simulink model "Rotary_inverted_pendulum_simscape_model"  (R2026b)
settings: Solver=VariableStepAuto  StopTime=10  EnableMultiTasking=on
InitFcn:
  | Rotary_inverted_pendulum_params;
values from neighbouring files (symbols this model uses):
  A = [0 0 1.58599833727e-11 -4.90689813272e-13 0 0 11.773740367 153.017565535 1 0 -0.668730280726 -0.988272810616 ... (16 elements, 4x4)]    [Rotary_inverted_pendulum_control_.mat]    (also in Rotary_inverted_pendulum_params.m = A_hand; Rotary_inverted_pendulum_symbolic.m = zeros(4,4))
  alpha_0 = 170    [Rotary_inverted_pendulum_params.m]
  alpha_cal = -3.678    [Rotary_inverted_pendulum_params.m]
  B = [0 0 3.48321726757 5.14775001613]    [Rotary_inverted_pendulum_control_.mat]    (also in Rotary_inverted_pendulum_params.m = B_hand; Rotary_inverted_pendulum_symbolic.m = zeros(4,1))
  C = [1 0 0 0; 0 1 0 0]    [Rotary_inverted_pendulum_params.m]
  D = [0; 0]    [Rotary_inverted_pendulum_params.m]
  K_c = place(A,B,[-8 -5 -6 -1])    [Rotary_inverted_pendulum_params.m]
  km = 0.035    [Rotary_inverted_pendulum_params.m]
  kt = 0.035    [Rotary_inverted_pendulum_params.m]
  L = 264e-6    (= 0.000264)    [Rotary_inverted_pendulum_params.m]
  L_o = place(A',C',5*[-8 -5 -6 -1])'    [Rotary_inverted_pendulum_params.m]
  link_mass = 0.08    [Rotary_inverted_pendulum_params.m]
  N = 1    [Rotary_inverted_pendulum_params.m]
  p_mass = 0.1    [Rotary_inverted_pendulum_params.m]
  R = 7.14    [Rotary_inverted_pendulum_params.m]    (also in Rotary_inverted_pendulum_symbolic.m = 2)
  rod_mass = 0.05    [Rotary_inverted_pendulum_params.m]
  rt1 = 7/2    (= 3.5)    [Rotary_inverted_pendulum_params.m]
  rt2 = 8.5-0.4    (= 8.1)    [Rotary_inverted_pendulum_params.m]
  V_max = 24    [Rotary_inverted_pendulum_params.m]
undefined symbols (not defined in the file or in its folder): K, L_q, X, Y, Z
libraries: sm_lib x123, nesl_utility x29, simulink x10
(part 1 of 4)
settings Model: Creator=ControlLab2  LastModifiedBy=Mrsh
settings DataIOCC: LimitDataPoints=on  MaxDataPoints=10000
settings OptimizationCC: LifeSpan=inf
settings DebuggingCC: AllowSymbolicDim=off  ArithmeticOperatorsInVariantConditions=warning  SFExecutionAtInitializationDiag=none  SFNoUnconditionalDefaultTransitionDiag=warning  SFUnexpectedBacktrackingDiag=warning
settings SFSimCC: CustomCodeUndefinedFunction=UseInterfaceOnly  SimUseLocalCustomCode=off
settings RTWCC: RTWUseLocalCustomCode=off
settings CodeAppCC: StateflowObjectComments=on
settings GRTTargetCC: TargetLangStandard=C89/C90 (ANSI)
settings ConfigComp: CovExternalEMLEnable=off  CovSFcnEnable=off  CovSaveCumulativeToWorkspaceVar=on  CovSaveSingleToWorkspaceVar=on
settings SimscapeCC: SimscapeLogSimulationStatistics=on  SimscapeLogType=all  SimscapeUseEnergyAccounting=off
settings ExplorerConfigSet: InternalSimMechanicsExplorerSettings=|
  | <ExplorerConfiguration>
  | 
  |   <canonicalview>default</canonicalview>
  | 
  |   <TilePanel>
  |     <TileInfo>
  |       <Tiles Columns="1" Count="1" Height="610" Rows="1" Width="1088">
  |         <Row Weight="1"/>
  |         <Column Weight="1"/>
  |         <Tile Height="1" Width="1" X="0" Y="0"/>
  |       </Tiles>
  |     </TileInfo>
  |     <SceneInfo>
  |       <SceneViewer>
  |         <IsThisViewStd>
  |           <IsStandardView>off</IsStandardView>
  |           <StandardViewName>Front</StandardViewName>
  |         </IsThisViewStd>
  |         <BGColor>
  |           <R>1</R>
  |           <G>1</G>
  |           <B>1</B>
  |           <A>1</A>
  |         </BGColor>
  |         <Camera>
  |           <DoPerspective>off</DoPerspective>
  |           <Position>
  |             <X>0.705670544528059</X>
  |             <Y>-0.69361970210692636</Y>
  |             <Z>0.40320052935287365</Z>
  |           </Position>
  |           <Center>
  |             <X>0.05090138860052084</X>
  |             <Y>-0.026375091476912745</Y>
  |             <Z>0.0012447022565247549</Z>
  |           </Center>
  |           <Up>
  |             <X>-0.2787747011801574</X>
  |             <Y>0.27985805213160481</Y>
  |             <Z>0.91867520737147246</Z>
  |           </Up>
  |           <XLim>0.14182089495266087</XLim>
  |           <YLim>0.14182089495266087</YLim>
  |           <ViewLimDist>0.01</ViewLimDist>
  |         </Camera>
  |       </SceneViewer>
  |     </SceneInfo>
  |   </TilePanel>
  | 
  |   <MechEditorPanel>
  |     <GfxPanelCameraMap/>
  |     <Cameras/>
  |     <VideoCreator>
  |       <IncludeTiles>All</IncludeTiles>
  |       <IncludeTime>on</IncludeTime>
  |       <IncludeWorldFrame>off</IncludeWorldFrame>
  |       <PlaybackSpeedRatio>1</PlaybackSpeedRatio>
  |       <FrameRate>30</FrameRate>
  |       <FrameSize>auto</FrameSize>
  |       <VideoFormat>MotionJPEGAVI</VideoFormat>
  |     </VideoCreator>
  |   </MechEditorPanel>
  | 
  |   <PlaybackSettings>
  |     <PlaybackSpeedFactor>1</PlaybackSpeedFactor>
  |   </PlaybackSettings>
  | 
  | </ExplorerConfiguration>

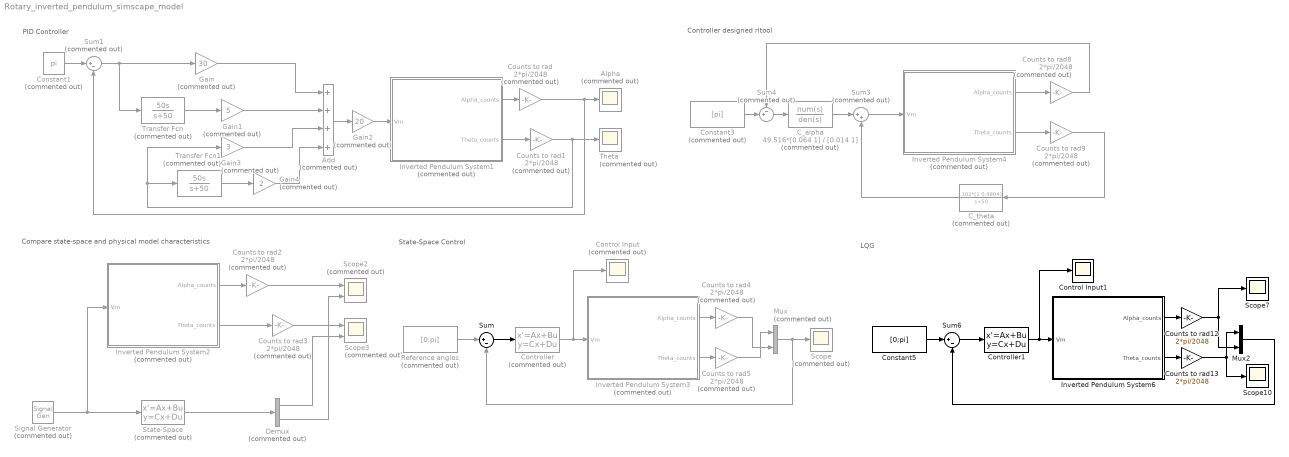
== system Rotary_inverted_pendulum_simscape_model ==
  note: PID Controller
  note: Compare state-space and physical model characteristics
  note: Controller designed rltool
  note: State-Space Control
  note: LQG
  Add : Sum  Commented=on  Inputs=++++
  Alpha : Scope  Commented=on
      settings: ActiveDisplayYMinimum=3.02651  ActiveDisplayYMaximum=3.22203
  C_alpha : TransferFcn  Commented=on  Numerator=49.516*[0.064 1]  Denominator=[0.014 1]
  C_theta : TransferFcn  Commented=on  Numerator=102*[1 0.9804]  Denominator=[1 50]
  Constant1 : Constant  Commented=on  Value=pi
  Constant3 : Constant  Commented=on  Value=[pi]
  Constant5 : Constant  Value=[0;pi]
  Control Input : Scope  Commented=on
      settings: ActiveDisplayYMinimum=-33.02101  ActiveDisplayYMaximum=31.32481
  Control Input1 : Scope
      settings: ActiveDisplayYMinimum=-7.48608  ActiveDisplayYMaximum=18.51296  DataLoggingVariableName=ULog  DataLoggingSaveFormat=Array
  Controller : StateSpace  Commented=on  A=A-B*K_c-L_o*C  B=L_o  C=K_c  D=[0 0]  InitialCondition=0
  Controller1 : StateSpace  A=A-B*K-L_q*C  B=L_q  C=K  D=[0 0]  InitialCondition=0
  Counts to rad{,1..5,8..9} (8 alike) : Gain  Commented=on  Gain=2*pi/2048
  Counts to rad12 : Gain  Gain=2*pi/2048
  Counts to rad13 : Gain  Gain=2*pi/2048
  Demux : Demux  Commented=on  Outputs=2
  Gain : Gain  Commented=on  Gain=30
  Gain1 : Gain  Commented=on  Gain=5
  Gain2 : Gain  Commented=on  Gain=20
  Gain3 : Gain  Commented=on  Gain=3
  Gain4 : Gain  Commented=on  Gain=2
  Inverted Pendulum System1 : Subsystem  Commented=on  mask{kt=kt, km=km, R=R, L=L, alpha_0=175}
      mask prompts: kt "Torque constant (Nm/A)"; km "Back EMF constant (V/(rad/s))"; R "Resistance (Ohm)"; L "Inductance (H)"; alpha_0 "Pendulum initial angle (deg)"
      mask init:
      | % Inverted Pendulum Parameters
      | base_size=7;%cm
      | rod_rad=1;
      | rod_length=8.5;
      | rod_mass=0.095;
      | p_rad=1;
      | p_length=12.9;
      | p_mass=0.024;
      | rt1=base_size/2;
      | rt2=rod_length-0.4;
      | rt4=p_length/2;
      | D_r=0.0015/2;
      | D_p=0.0005/2;
  Inverted Pendulum System2 : Subsystem  Commented=on  mask{kt=kt, km=km, R=R, L=L, alpha_0=0}
      mask prompts: kt "Torque constant (Nm/A)"; km "Back EMF constant (V/(rad/s))"; R "Resistance (Ohm)"; L "Inductance (H)"; alpha_0 "Pendulum initial angle (deg)"
      mask init: same as Rotary_inverted_pendulum_simscape_model/Inverted Pendulum System1
  Inverted Pendulum System3 : Subsystem  Commented=on  mask{kt=kt, km=km, R=R, L=L, alpha_0=165}
      mask prompts: kt "Torque constant (Nm/A)"; km "Back EMF constant (V/(rad/s))"; R "Resistance (Ohm)"; L "Inductance (H)"; alpha_0 "Pendulum initial angle (deg)"
      mask init: same as Rotary_inverted_pendulum_simscape_model/Inverted Pendulum System1
  Inverted Pendulum System4 : Subsystem  Commented=on  mask{kt=kt, km=km, R=R, L=L, alpha_0=175}
      mask prompts: kt "Torque constant (Nm/A)"; km "Back EMF constant (V/(rad/s))"; R "Resistance (Ohm)"; L "Inductance (H)"; alpha_0 "Pendulum initial angle (deg)"
      mask init: same as Rotary_inverted_pendulum_simscape_model/Inverted Pendulum System1
  Inverted Pendulum System6 : Subsystem  mask{kt=kt, km=km, R=R, L=L, alpha_0=alpha_0}
      mask prompts: kt "Torque constant (Nm/A)"; km "Back EMF constant (V/(rad/s))"; R "Resistance (Ohm)"; L "Inductance (H)"; alpha_0 "Pendulum initial angle (deg)"
      mask init:
      | % All parameters come from Rotary_inverted_pendulum_realistic_params.m
  Mux : Mux  Commented=on  Inputs=2
  Mux2 : Mux  Inputs=2
  Reference angles : Constant  Commented=on  Value=[0;pi]
  Scope : Scope  Commented=on
      settings: ActiveDisplayYMinimum=-0.50694  ActiveDisplayYMaximum=3.69747  DataLoggingVariableName=ScopeData3
  Scope10 : Scope
      settings: ActiveDisplayYMinimum=-0.24263  ActiveDisplayYMaximum=1.50161  DataLoggingVariableName=ThetaLog  DataLoggingSaveFormat=Array
  Scope2 : Scope  Commented=on  NumInputPorts=2
      settings: ActiveDisplayYMinimum=-4.48254  ActiveDisplayYMaximum=4.62282  DataLoggingVariableName=ScopeData2
  Scope3 : Scope  Commented=on  NumInputPorts=2
      settings: ActiveDisplayYMinimum=-8.30374  ActiveDisplayYMaximum=0.94912  DataLoggingVariableName=ScopeData3
  Scope7 : Scope
      settings: ActiveDisplayYMinimum=2.818  ActiveDisplayYMaximum=3.3143  DataLoggingVariableName=AlphaLog  DataLoggingSaveFormat=Array
  Signal Generator : SignalGenerator  Commented=on  WaveForm=square
  State-Space : StateSpace  Commented=on  A=A  B=B  C=C  D=D  InitialCondition=0
  Sum : Sum  Inputs=|+-
  Sum1 : Sum  Commented=on  Inputs=|+-
  Sum3 : Sum  Commented=on  Inputs=|++
  Sum4 : Sum  Commented=on  Inputs=-+|
  Sum6 : Sum  Inputs=|+-
  Theta : Scope  Commented=on
      settings: ActiveDisplayYMinimum=-0.10248  ActiveDisplayYMaximum=0.25695  DataLoggingVariableName=ScopeData2
  Transfer Fcn : TransferFcn  Commented=on  Numerator=[50 0]  Denominator=[1 50]
  Transfer Fcn1 : TransferFcn  Commented=on  Numerator=[50 0]  Denominator=[1 50]
  wires:
  Constant1/1 -> Sum1/1
  Inverted Pendulum System1/1(Alpha_counts) -> Counts to rad/1
  Transfer Fcn/1 -> Gain1/1
  Transfer Fcn1/1 -> Gain4/1
  Inverted Pendulum System1/2(Theta_counts) -> Counts to rad1/1
  Gain/1 -> Add/1
  Gain1/1 -> Add/2
  Gain3/1 -> Add/3
  Gain4/1 -> Add/4
  Add/1 -> Gain2/1
  Signal Generator/1 -> Inverted Pendulum System2/1(Vm), State-Space/1
  Sum1/1 -> Transfer Fcn/1, Gain/1
  Inverted Pendulum System2/1(Alpha_counts) -> Counts to rad2/1
  Inverted Pendulum System2/2(Theta_counts) -> Counts to rad3/1
  Gain2/1 -> Inverted Pendulum System1/1(Vm)
  State-Space/1 -> Demux/1
  Demux/1 -> Scope3/2
  Demux/2 -> Scope2/2
  Reference angles/1 -> Sum/1
  Sum/1 -> Controller/1
  Mux/1 -> Scope/1, Sum/2
  Inverted Pendulum System3/2(Theta_counts) -> Counts to rad5/1
  Inverted Pendulum System3/1(Alpha_counts) -> Counts to rad4/1
  Counts to rad/1 -> Alpha/1, Sum1/2
  Counts to rad1/1 -> Theta/1, Transfer Fcn1/1, Gain3/1
  Counts to rad2/1 -> Scope2/1
  Counts to rad3/1 -> Scope3/1
  Counts to rad4/1 -> Mux/2
  Counts to rad5/1 -> Mux/1
  Controller/1 -> Inverted Pendulum System3/1(Vm), Control Input/1
  Inverted Pendulum System4/2(Theta_counts) -> Counts to rad9/1
  Inverted Pendulum System4/1(Alpha_counts) -> Counts to rad8/1
  C_theta/1 -> Sum3/2
  Counts to rad9/1 -> C_theta/1
  Constant3/1 -> Sum4/2
  Counts to rad8/1 -> Sum4/1
  Sum4/1 -> C_alpha/1
  C_alpha/1 -> Sum3/1
  Sum3/1 -> Inverted Pendulum System4/1(Vm)
  Controller1/1 -> Inverted Pendulum System6/1(Vm), Control Input1/1
  Constant5/1 -> Sum6/1
  Mux2/1 -> Sum6/2
  Inverted Pendulum System6/2(Theta_counts) -> Counts to rad13/1
  Inverted Pendulum System6/1(Alpha_counts) -> Counts to rad12/1
  Sum6/1 -> Controller1/1
  Counts to rad13/1 -> Scope10/1, Mux2/1
  Counts to rad12/1 -> Scope7/1, Mux2/2

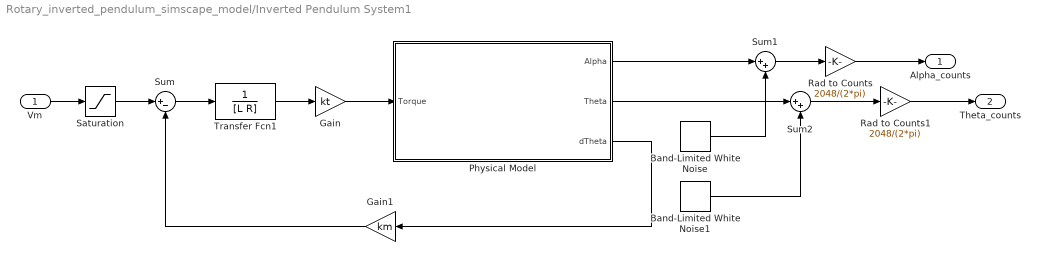
== system Rotary_inverted_pendulum_simscape_model/Inverted Pendulum System1 ==
  Vm : Inport
  Band-Limited White Noise : simulink/Sources/Band-Limited White Noise  Cov=[0.0000001]  Ts=0.001  seed=[23341]
  Band-Limited White Noise1 : simulink/Sources/Band-Limited White Noise  Cov=[0.0000001]  Ts=0.001  seed=[23341]
  Gain : Gain  Gain=kt
  Gain1 : Gain  Gain=km
  Physical Model : Subsystem
  Rad to Counts : Gain  Gain=2048/(2*pi)
  Rad to Counts1 : Gain  Gain=2048/(2*pi)
  Saturation : Saturate  UpperLimit=10  LowerLimit=-10
  Sum : Sum  Inputs=|+-
  Sum1 : Sum  Inputs=|++
  Sum2 : Sum  Inputs=|++
  Transfer Fcn1 : TransferFcn  Denominator=[L R]
  Alpha_counts : Outport
  Theta_counts : Outport  Port=2
  wires:
  Saturation/1 -> Sum/1
  Rad to Counts1/1 -> Theta_counts/1
  Rad to Counts/1 -> Alpha_counts/1
  Band-Limited White Noise1/1 -> Sum2/2
  Band-Limited White Noise/1 -> Sum1/2
  Sum2/1 -> Rad to Counts1/1
  Sum1/1 -> Rad to Counts/1
  Sum/1 -> Transfer Fcn1/1
  Transfer Fcn1/1 -> Gain/1
  Gain1/1 -> Sum/2
  Physical Model/3(dTheta) -> Gain1/1
  Gain/1 -> Physical Model/1(Torque)
  Vm/1 -> Saturation/1
  Physical Model/1(Alpha) -> Sum1/1
  Physical Model/2(Theta) -> Sum2/1

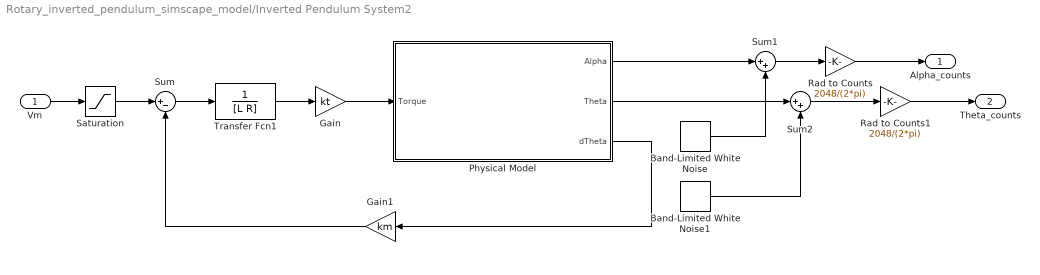
== system Rotary_inverted_pendulum_simscape_model/Inverted Pendulum System2 ==
  Vm : Inport
  Band-Limited White Noise : simulink/Sources/Band-Limited White Noise  Cov=[0.0000001]  Ts=0.001  seed=[23341]
  Band-Limited White Noise1 : simulink/Sources/Band-Limited White Noise  Cov=[0.0000001]  Ts=0.001  seed=[23341]
  Gain : Gain  Gain=kt
  Gain1 : Gain  Gain=km
  Physical Model : Subsystem
  Rad to Counts : Gain  Gain=2048/(2*pi)
  Rad to Counts1 : Gain  Gain=2048/(2*pi)
  Saturation : Saturate  UpperLimit=10  LowerLimit=-10
  Sum : Sum  Inputs=|+-
  Sum1 : Sum  Inputs=|++
  Sum2 : Sum  Inputs=|++
  Transfer Fcn1 : TransferFcn  Denominator=[L R]
  Alpha_counts : Outport
  Theta_counts : Outport  Port=2
  wires:
  Saturation/1 -> Sum/1
  Rad to Counts1/1 -> Theta_counts/1
  Rad to Counts/1 -> Alpha_counts/1
  Band-Limited White Noise1/1 -> Sum2/2
  Band-Limited White Noise/1 -> Sum1/2
  Sum2/1 -> Rad to Counts1/1
  Sum1/1 -> Rad to Counts/1
  Sum/1 -> Transfer Fcn1/1
  Transfer Fcn1/1 -> Gain/1
  Gain1/1 -> Sum/2
  Physical Model/3(dTheta) -> Gain1/1
  Gain/1 -> Physical Model/1(Torque)
  Vm/1 -> Saturation/1
  Physical Model/1(Alpha) -> Sum1/1
  Physical Model/2(Theta) -> Sum2/1

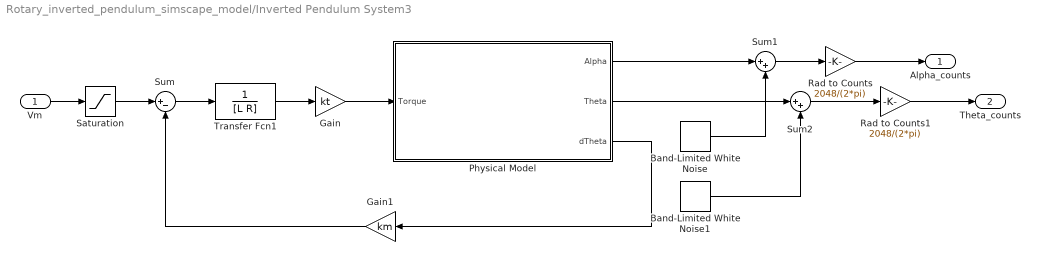
== system Rotary_inverted_pendulum_simscape_model/Inverted Pendulum System3 ==
  Vm : Inport
  Band-Limited White Noise : simulink/Sources/Band-Limited White Noise  Cov=[0.0000001]  Ts=0.001  seed=[23341]
  Band-Limited White Noise1 : simulink/Sources/Band-Limited White Noise  Cov=[0.0000001]  Ts=0.001  seed=[23341]
  Gain : Gain  Gain=kt
  Gain1 : Gain  Gain=km
  Physical Model : Subsystem
  Rad to Counts : Gain  Gain=2048/(2*pi)
  Rad to Counts1 : Gain  Gain=2048/(2*pi)
  Saturation : Saturate  UpperLimit=10  LowerLimit=-10
  Sum : Sum  Inputs=|+-
  Sum1 : Sum  Inputs=|++
  Sum2 : Sum  Inputs=|++
  Transfer Fcn1 : TransferFcn  Denominator=[L R]
  Alpha_counts : Outport
  Theta_counts : Outport  Port=2
  wires:
  Saturation/1 -> Sum/1
  Rad to Counts1/1 -> Theta_counts/1
  Rad to Counts/1 -> Alpha_counts/1
  Band-Limited White Noise1/1 -> Sum2/2
  Band-Limited White Noise/1 -> Sum1/2
  Sum2/1 -> Rad to Counts1/1
  Sum1/1 -> Rad to Counts/1
  Sum/1 -> Transfer Fcn1/1
  Transfer Fcn1/1 -> Gain/1
  Gain1/1 -> Sum/2
  Physical Model/3(dTheta) -> Gain1/1
  Gain/1 -> Physical Model/1(Torque)
  Vm/1 -> Saturation/1
  Physical Model/1(Alpha) -> Sum1/1
  Physical Model/2(Theta) -> Sum2/1

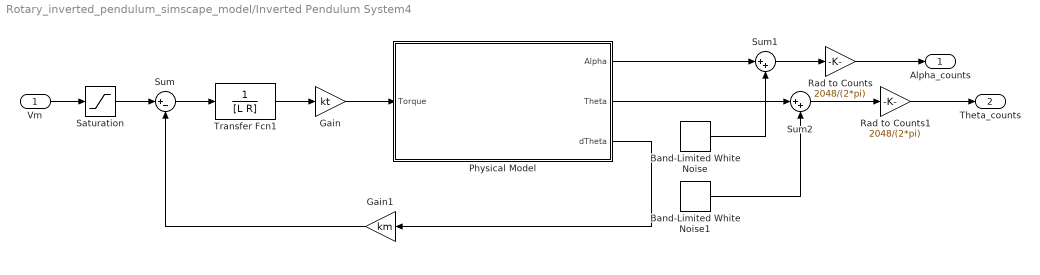
== system Rotary_inverted_pendulum_simscape_model/Inverted Pendulum System4 ==
  Vm : Inport
  Band-Limited White Noise : simulink/Sources/Band-Limited White Noise  Cov=[0.0000001]  Ts=0.001  seed=[23341]
  Band-Limited White Noise1 : simulink/Sources/Band-Limited White Noise  Cov=[0.0000001]  Ts=0.001  seed=[23341]
  Gain : Gain  Gain=kt
  Gain1 : Gain  Gain=km
  Physical Model : Subsystem
  Rad to Counts : Gain  Gain=2048/(2*pi)
  Rad to Counts1 : Gain  Gain=2048/(2*pi)
  Saturation : Saturate  UpperLimit=10  LowerLimit=-10
  Sum : Sum  Inputs=|+-
  Sum1 : Sum  Inputs=|++
  Sum2 : Sum  Inputs=|++
  Transfer Fcn1 : TransferFcn  Denominator=[L R]
  Alpha_counts : Outport
  Theta_counts : Outport  Port=2
  wires:
  Saturation/1 -> Sum/1
  Rad to Counts1/1 -> Theta_counts/1
  Rad to Counts/1 -> Alpha_counts/1
  Band-Limited White Noise1/1 -> Sum2/2
  Band-Limited White Noise/1 -> Sum1/2
  Sum2/1 -> Rad to Counts1/1
  Sum1/1 -> Rad to Counts/1
  Sum/1 -> Transfer Fcn1/1
  Transfer Fcn1/1 -> Gain/1
  Gain1/1 -> Sum/2
  Physical Model/3(dTheta) -> Gain1/1
  Gain/1 -> Physical Model/1(Torque)
  Vm/1 -> Saturation/1
  Physical Model/1(Alpha) -> Sum1/1
  Physical Model/2(Theta) -> Sum2/1

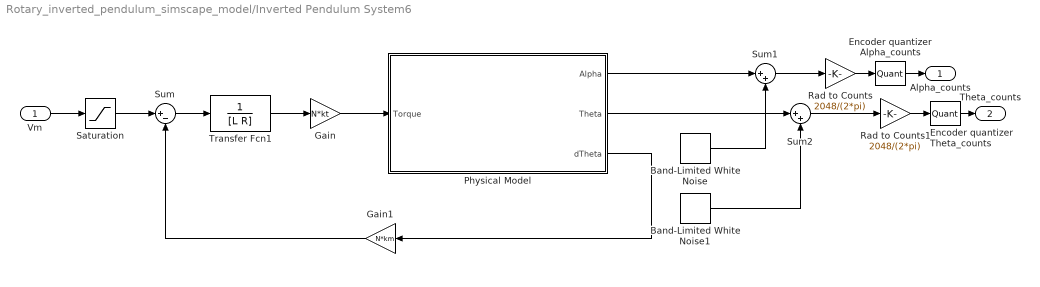
== system Rotary_inverted_pendulum_simscape_model/Inverted Pendulum System6 ==
  Vm : Inport
  Band-Limited White Noise : simulink/Sources/Band-Limited White Noise  Cov=[0.0000001]  Ts=0.001  seed=[23341]
  Band-Limited White Noise1 : simulink/Sources/Band-Limited White Noise  Cov=[0.0000001]  Ts=0.001  seed=[23341]
  Encoder quantizer Alpha_counts : Quantizer  QuantizationInterval=1
  Encoder quantizer Theta_counts : Quantizer  QuantizationInterval=1
  Gain : Gain  Gain=N*kt
  Gain1 : Gain  Gain=N*km
  Physical Model : Subsystem
  Rad to Counts : Gain  Gain=2048/(2*pi)
  Rad to Counts1 : Gain  Gain=2048/(2*pi)
  Saturation : Saturate  UpperLimit=V_max  LowerLimit=-V_max
  Sum : Sum  Inputs=|+-
  Sum1 : Sum  Inputs=|++
  Sum2 : Sum  Inputs=|++
  Transfer Fcn1 : TransferFcn  Denominator=[L R]
  Alpha_counts : Outport
  Theta_counts : Outport  Port=2
  wires:
  Saturation/1 -> Sum/1
  Band-Limited White Noise1/1 -> Sum2/2
  Band-Limited White Noise/1 -> Sum1/2
  Sum2/1 -> Rad to Counts1/1
  Sum1/1 -> Rad to Counts/1
  Sum/1 -> Transfer Fcn1/1
  Transfer Fcn1/1 -> Gain/1
  Gain1/1 -> Sum/2
  Physical Model/3(dTheta) -> Gain1/1
  Gain/1 -> Physical Model/1(Torque)
  Vm/1 -> Saturation/1
  Physical Model/1(Alpha) -> Sum1/1
  Physical Model/2(Theta) -> Sum2/1
  Rad to Counts/1 -> Encoder quantizer Alpha_counts/1
  Encoder quantizer Alpha_counts/1 -> Alpha_counts/1
  Rad to Counts1/1 -> Encoder quantizer Theta_counts/1
  Encoder quantizer Theta_counts/1 -> Theta_counts/1

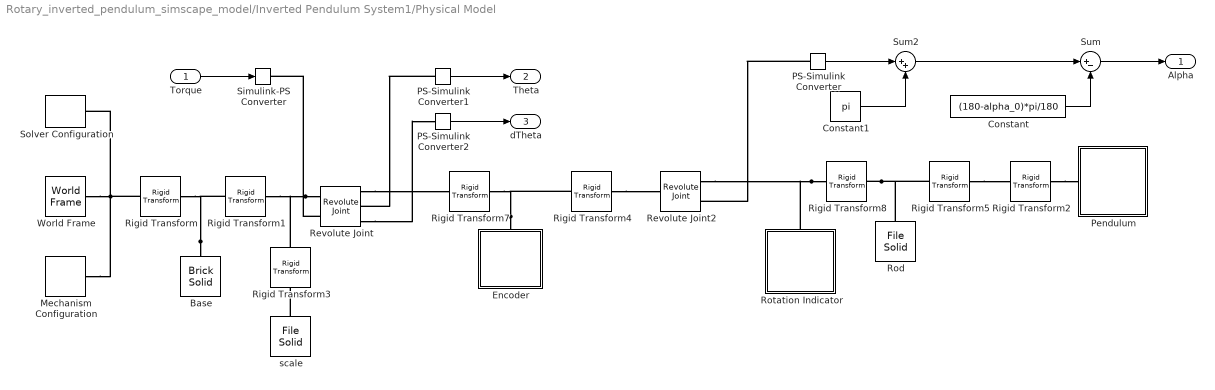
== system Rotary_inverted_pendulum_simscape_model/Inverted Pendulum System1/Physical Model ==
  Torque : Inport
  Base : sm_lib/Body Elements/Brick Solid  GraphicAmbientColor=[0.15 0.15 0.15 1.0]  BasedOnType=Density  BrickDimensions=[1 1 1]*base_size  BrickDimensionUnits=cm  CenterOfMass=[0 0 0]  CenterOfMassUnits=m  GraphicDiffuseColor=[0.4 0.4 0.4]  Density=1000  DensityUnits=kg/m^3  DoExposeReferenceFrame=on  GraphicEmissiveColor=[0.0 0.0 0.0 1.0]  ExportEntireGeometry=off  SerializedFrames=<Frames/>  MarkerShape=Sphere  MarkerSize=10  GraphicType=FromGeometry  InertiaType=CalculateFromGeometry  Mass=1  MassUnits=kg  MomentsOfInertia=[1 1 1]  MomentsOfInertiaUnits=kg*m^2  GraphicOpacity=1.0  ProductsOfInertia=[0 0 0]  ProductsOfInertiaUnits=kg*m^2  GraphicShininess=75  GraphicSpecularColor=[0.5 0.5 0.5 1.0]  GraphicVisPropType=SimpleVisualProperties
  Constant : Constant  Value=(180-alpha_0)*pi/180
  Constant1 : Constant  Value=pi
  Encoder : Subsystem
  Mechanism Configuration : sm_lib/Utilities/Mechanism Configuration  UniformGravity=Constant  GravityVector=[0 0 -9.80665]  GravityUnits=m/s^2  LinearizationDelta=0.001
  PS-Simulink Converter : nesl_utility/PS-Simulink Converter  PhysicalDomain=network_engine_domain  SubClassName=ps_output  LeftPortType=input  RightPortType=output  PseudoPeriodic=off  Frequencies=[]  Unit=inherit  AffineConversion=off
  PS-Simulink Converter1 : nesl_utility/PS-Simulink Converter  PhysicalDomain=network_engine_domain  SubClassName=ps_output  LeftPortType=input  RightPortType=output  PseudoPeriodic=off  Frequencies=[]  Unit=inherit  AffineConversion=off
  PS-Simulink Converter2 : nesl_utility/PS-Simulink Converter  PhysicalDomain=network_engine_domain  SubClassName=ps_output  LeftPortType=input  RightPortType=output  PseudoPeriodic=off  Frequencies=[]  Unit=inherit  AffineConversion=off
  Pendulum : Subsystem
  Revolute Joint : sm_lib/Joints/Revolute Joint  JointMode=Normal  SenseConstraintForce=off  SenseConstraintForceX=off  SenseConstraintForceY=off  SenseConstraintForceZ=off  SenseConstraintTorque=off  SenseConstraintTorqueX=off  SenseConstraintTorqueY=off  SenseConstraintTorqueZ=off  SenseTotalForce=off  SenseTotalForceX=off  SenseTotalForceY=off  SenseTotalForceZ=off  SenseTotalTorque=off  SenseTotalTorqueX=off  SenseTotalTorqueY=off  SenseTotalTorqueZ=off  CompositeWrenchDir=FollowerOnBase  CompositeWrenchFrame=BaseFrame  EquilibriumPosition=0  EquilibriumPositionUnits=deg  SpringStiffness=0  SpringStiffnessUnits=N*m/deg  DampingCoefficient=D_r  DampingCoefficientUnits=N*m/(rad/s)  TorqueActuationMode=InputTorque  MotionActuationMode=ComputedMotion  SensePosition=on  SenseVelocity=on  SenseAcceleration=off  SenseTorqueForce=off  SenseLowerLimitTorqueForce=off  SenseUpperLimitTorqueForce=off  LowerLimitSpecify=off  LowerLimitBound=-90  LowerLimitBoundUnits=deg  LowerLimitStiffness=1e4  LowerLimitStiffnessUnits=N*m/deg  LowerLimitDamping=10  LowerLimitDampingUnits=N*m/(deg/s)  LowerLimitTransitionRegionWidth=0.1  LowerLimitTransitionRegionWidthUnits=deg  UpperLimitSpecify=off  UpperLimitBound=90  UpperLimitBoundUnits=deg  UpperLimitStiffness=1e4  UpperLimitStiffnessUnits=N*m/deg  UpperLimitDamping=10  UpperLimitDampingUnits=N*m/(deg/s)  UpperLimitTransitionRegionWidth=0.1  UpperLimitTransitionRegionWidthUnits=deg  PositionTargetSpecify=off  PositionTargetPriority=High  PositionTargetValue=0  PositionTargetValueUnits=deg  VelocityTargetSpecify=off  VelocityTargetPriority=High  VelocityTargetValue=0  VelocityTargetValueUnits=deg/s
  Revolute Joint2 : sm_lib/Joints/Revolute Joint  JointMode=Normal  SenseConstraintForce=off  SenseConstraintForceX=off  SenseConstraintForceY=off  SenseConstraintForceZ=off  SenseConstraintTorque=off  SenseConstraintTorqueX=off  SenseConstraintTorqueY=off  SenseConstraintTorqueZ=off  SenseTotalForce=off  SenseTotalForceX=off  SenseTotalForceY=off  SenseTotalForceZ=off  SenseTotalTorque=off  SenseTotalTorqueX=off  SenseTotalTorqueY=off  SenseTotalTorqueZ=off  CompositeWrenchDir=FollowerOnBase  CompositeWrenchFrame=BaseFrame  EquilibriumPosition=0  EquilibriumPositionUnits=deg  SpringStiffness=0  SpringStiffnessUnits=N*m/deg  DampingCoefficient=D_p  DampingCoefficientUnits=N*m/(rad/s)  TorqueActuationMode=NoTorque  MotionActuationMode=ComputedMotion  SensePosition=on  SenseVelocity=off  SenseAcceleration=off  SenseTorqueForce=off  SenseLowerLimitTorqueForce=off  SenseUpperLimitTorqueForce=off  LowerLimitSpecify=off  LowerLimitBound=-90  LowerLimitBoundUnits=deg  LowerLimitStiffness=1e4  LowerLimitStiffnessUnits=N*m/deg  LowerLimitDamping=10  LowerLimitDampingUnits=N*m/(deg/s)  LowerLimitTransitionRegionWidth=0.1  LowerLimitTransitionRegionWidthUnits=deg  UpperLimitSpecify=off  UpperLimitBound=90  UpperLimitBoundUnits=deg  UpperLimitStiffness=1e4  UpperLimitStiffnessUnits=N*m/deg  UpperLimitDamping=10  UpperLimitDampingUnits=N*m/(deg/s)  UpperLimitTransitionRegionWidth=0.1  UpperLimitTransitionRegionWidthUnits=deg  PositionTargetSpecify=off  PositionTargetPriority=High  PositionTargetValue=0  PositionTargetValueUnits=deg  VelocityTargetSpecify=off  VelocityTargetPriority=High  VelocityTargetValue=0  VelocityTargetValueUnits=deg/s
  Rigid Transform : sm_lib/Frames and Transforms/Rigid Transform  TranslationMethod=None  TranslationStandardOffset=0  TranslationLengthUnit=m  TranslationStandardAxis=+Z  TranslationCartesianOffset=[0 0 0]  TranslationROffset=0  TranslationROffsetUnits=m  TranslationZOffset=0  TranslationZOffsetUnits=m  TranslationThetaOffset=0  TranslationThetaOffsetUnits=deg  RotationMethod=None  RotationAngleUnits=deg  RotationStandardAxis=+Z  RotationAngle=0.0  RotationArbitraryAxis=[0 0 1]  FollAlignAxisA=+X  BaseAlignAxisA=+Y  FollAlignAxisB=+Y  BaseAlignAxisB=+Z  RotationSequenceAxes=FollowerAxes  RotationSequence=XYX  RotationSequenceAngles=[0 0 0]  RotationSequenceAnglesUnits=deg  RotationMatrix=[1 0 0; 0 1 0; 0 0 1]
  Rigid Transform1 : sm_lib/Frames and Transforms/Rigid Transform  TranslationMethod=Cartesian  TranslationStandardOffset=0  TranslationLengthUnit=cm  TranslationStandardAxis=+Z  TranslationCartesianOffset=[0 0 rt1]  TranslationROffset=0  TranslationROffsetUnits=m  TranslationZOffset=0  TranslationZOffsetUnits=m  TranslationThetaOffset=0  TranslationThetaOffsetUnits=deg  RotationMethod=None  RotationAngleUnits=deg  RotationStandardAxis=+Y  RotationAngle=90  RotationArbitraryAxis=[0 0 1]  FollAlignAxisA=+X  BaseAlignAxisA=+Y  FollAlignAxisB=+Y  BaseAlignAxisB=+Z  RotationSequenceAxes=FollowerAxes  RotationSequence=XYX  RotationSequenceAngles=[0 0 0]  RotationSequenceAnglesUnits=deg  RotationMatrix=[1 0 0; 0 1 0; 0 0 1]
  Rigid Transform2 : sm_lib/Frames and Transforms/Rigid Transform  TranslationMethod=Cartesian  TranslationStandardOffset=0  TranslationLengthUnit=cm  TranslationStandardAxis=+Z  TranslationCartesianOffset=[0 0 rt2]  TranslationROffset=0  TranslationROffsetUnits=m  TranslationZOffset=0  TranslationZOffsetUnits=m  TranslationThetaOffset=0  TranslationThetaOffsetUnits=deg  RotationMethod=None  RotationAngleUnits=deg  RotationStandardAxis=+Y  RotationAngle=90  RotationArbitraryAxis=[0 0 1]  FollAlignAxisA=+X  BaseAlignAxisA=+Y  FollAlignAxisB=+Y  BaseAlignAxisB=+Z  RotationSequenceAxes=FollowerAxes  RotationSequence=XYX  RotationSequenceAngles=[0 0 0]  RotationSequenceAnglesUnits=deg  RotationMatrix=[1 0 0; 0 1 0; 0 0 1]
  Rigid Transform3 : sm_lib/Frames and Transforms/Rigid Transform  TranslationMethod=None  TranslationStandardOffset=0  TranslationLengthUnit=cm  TranslationStandardAxis=+Z  TranslationCartesianOffset=[0 0 rt1]  TranslationROffset=0  TranslationROffsetUnits=m  TranslationZOffset=0  TranslationZOffsetUnits=m  TranslationThetaOffset=0  TranslationThetaOffsetUnits=deg  RotationMethod=RotationSequence  RotationAngleUnits=deg  RotationStandardAxis=+X  RotationAngle=90  RotationArbitraryAxis=[0 0 1]  FollAlignAxisA=+X  BaseAlignAxisA=+Y  FollAlignAxisB=+Y  BaseAlignAxisB=+Z  RotationSequenceAxes=FollowerAxes  RotationSequence=XYX  RotationSequenceAngles=[90 -90 0]  RotationSequenceAnglesUnits=deg  RotationMatrix=[1 0 0; 0 1 0; 0 0 1]
  Rigid Transform4 : sm_lib/Frames and Transforms/Rigid Transform  TranslationMethod=Cartesian  TranslationStandardOffset=0  TranslationLengthUnit=cm  TranslationStandardAxis=+Z  TranslationCartesianOffset=[-1.3 1 0]  TranslationROffset=0  TranslationROffsetUnits=m  TranslationZOffset=0  TranslationZOffsetUnits=m  TranslationThetaOffset=0  TranslationThetaOffsetUnits=deg  RotationMethod=StandardAxis  RotationAngleUnits=deg  RotationStandardAxis=+Y  RotationAngle=90  RotationArbitraryAxis=[0 0 1]  FollAlignAxisA=+X  BaseAlignAxisA=+Y  FollAlignAxisB=+Y  BaseAlignAxisB=+Z  RotationSequenceAxes=FollowerAxes  RotationSequence=XYX  RotationSequenceAngles=[0 0 0]  RotationSequenceAnglesUnits=deg  RotationMatrix=[1 0 0; 0 1 0; 0 0 1]
  Rigid Transform5 : sm_lib/Frames and Transforms/Rigid Transform  TranslationMethod=None  TranslationStandardOffset=0  TranslationLengthUnit=cm  TranslationStandardAxis=+Z  TranslationCartesianOffset=[0 0 rt2]  TranslationROffset=0  TranslationROffsetUnits=m  TranslationZOffset=0  TranslationZOffsetUnits=m  TranslationThetaOffset=0  TranslationThetaOffsetUnits=deg  RotationMethod=StandardAxis  RotationAngleUnits=deg  RotationStandardAxis=+Y  RotationAngle=90  RotationArbitraryAxis=[0 0 1]  FollAlignAxisA=+X  BaseAlignAxisA=+Y  FollAlignAxisB=+Y  BaseAlignAxisB=+Z  RotationSequenceAxes=FollowerAxes  RotationSequence=XYX  RotationSequenceAngles=[0 0 0]  RotationSequenceAnglesUnits=deg  RotationMatrix=[1 0 0; 0 1 0; 0 0 1]
  Rigid Transform7 : sm_lib/Frames and Transforms/Rigid Transform  TranslationMethod=Cartesian  TranslationStandardOffset=0  TranslationLengthUnit=cm  TranslationStandardAxis=+Z  TranslationCartesianOffset=[0 0 0.5]  TranslationROffset=0  TranslationROffsetUnits=m  TranslationZOffset=0  TranslationZOffsetUnits=m  TranslationThetaOffset=0  TranslationThetaOffsetUnits=deg  RotationMethod=StandardAxis  RotationAngleUnits=deg  RotationStandardAxis=+X  RotationAngle=90  RotationArbitraryAxis=[0 0 1]  FollAlignAxisA=+X  BaseAlignAxisA=+Y  FollAlignAxisB=+Y  BaseAlignAxisB=+Z  RotationSequenceAxes=FollowerAxes  RotationSequence=XYX  RotationSequenceAngles=[0 0 0]  RotationSequenceAnglesUnits=deg  RotationMatrix=[1 0 0; 0 1 0; 0 0 1]
  Rigid Transform8 : sm_lib/Frames and Transforms/Rigid Transform  TranslationMethod=None  TranslationStandardOffset=0  TranslationLengthUnit=cm  TranslationStandardAxis=+Z  TranslationCartesianOffset=[-1.3 1 0]  TranslationROffset=0  TranslationROffsetUnits=m  TranslationZOffset=0  TranslationZOffsetUnits=m  TranslationThetaOffset=0  TranslationThetaOffsetUnits=deg  RotationMethod=StandardAxis  RotationAngleUnits=deg  RotationStandardAxis=+Y  RotationAngle=-90  RotationArbitraryAxis=[0 0 1]  FollAlignAxisA=+X  BaseAlignAxisA=+Y  FollAlignAxisB=+Y  BaseAlignAxisB=+Z  RotationSequenceAxes=FollowerAxes  RotationSequence=XYX  RotationSequenceAngles=[0 0 0]  RotationSequenceAnglesUnits=deg  RotationMatrix=[1 0 0; 0 1 0; 0 0 1]
  Rod : sm_lib/Body Elements/File Solid  ExtGeomFileName=step_rod.STEP  UnitType=FromFile  ExtGeomFileUnits=cm  StepReaderType=HEX  ExportEntireGeometry=off  InertiaType=CalculateFromGeometry  Mass=rod_mass  MassUnits=kg  CenterOfMass=[0 0 0]  CenterOfMassUnits=m  MomentsOfInertia=[1 1 1]  MomentsOfInertiaUnits=kg*m^2  ProductsOfInertia=[0 0 0]  ProductsOfInertiaUnits=kg*m^2  BasedOnType=Mass  Density=1000  DensityUnits=kg/m^3  DoExposeReferenceFrame=on  SerializedFrames=<Frames/>  GraphicType=FromGeometry  MarkerShape=Frame  MarkerSize=10  GraphicVisPropType=FromFileVisualProperties  GraphicDiffuseColor=[0.5 0.5 0.5]  GraphicSpecularColor=[0.5 0.5 0.5 1.0]  GraphicAmbientColor=[0.15 0.15 0.15 1.0]  GraphicEmissiveColor=[0.0 0.0 0.0 1.0]  GraphicShininess=75  GraphicOpacity=1.0
  Rotation Indicator : Subsystem
  Simulink-PS Converter : nesl_utility/Simulink-PS Converter  PhysicalDomain=network_engine_domain  SubClassName=ps_input  LeftPortType=input  RightPortType=output  PseudoPeriodic=off  Frequencies=[]  NoiseDistribution=none  NoiseParameters=[]  Unit=1  AffineConversion=off  FilteringAndDerivatives=provide  SimscapeFilterOrder=1  InputFilterTimeConstant=0.001  UdotUserProvided=0
  Solver Configuration : nesl_utility/Solver Configuration  PhysicalDomain=network_engine_domain  SubClassName=solver  LeftPortType=input  RightPortType=generic  Tones=[]  Harmonics=[]  SimulateNoise=off  Profile=off  UseLocalSampling=off  EnableSwitchedLinearOptims=on  FrequencyDomain=off  UseCCode=off  RelTol=0.001  AbsTol=1e-06  MinStep=1e-09  ToWorkspace=off  RevertToSquareIcSolve=off  NumHomotopyIterations=100  PhasorMode=off  PhasorModeNumHarmonics=1  DoDC=off  ResidualTolerance=1e-09  UseLocalSolver=off  LocalSolverChoice=NE_BACKWARD_EULER_ADVANCER  LocalSolverSampleTime=0.001  DoFixedCost=off  MaxNonlinIter=3  MaxModeIter=2  LinearAlgebra=Sparse  EquationFormulation=NE_TIME_EF  DelaysMemoryBudget=1024  AutomaticFiltering=on  FilteringTimeConstant=0.001  PartitionStorageMethod=AS_NEEDED  PartitionMemoryBudget=1024  PartitionMethod=FAST
  Sum : Sum  Inputs=|+-
  Sum2 : Sum  Inputs=|++
  World Frame : sm_lib/Frames and Transforms/World Frame
  scale : sm_lib/Body Elements/File Solid  ExtGeomFileName=step_angles.STEP  UnitType=FromFile  ExtGeomFileUnits=cm  StepReaderType=HEX  ExportEntireGeometry=off  InertiaType=CalculateFromGeometry  Mass=rod_mass  MassUnits=kg  CenterOfMass=[0 0 0]  CenterOfMassUnits=m  MomentsOfInertia=[1 1 1]  MomentsOfInertiaUnits=kg*m^2  ProductsOfInertia=[0 0 0]  ProductsOfInertiaUnits=kg*m^2  BasedOnType=Mass  Density=1000  DensityUnits=kg/m^3  DoExposeReferenceFrame=on  SerializedFrames=<Frames/>  GraphicType=FromGeometry  MarkerShape=Frame  MarkerSize=10  GraphicVisPropType=SimpleVisualProperties  GraphicDiffuseColor=[1.0 1.0 1.0]  GraphicSpecularColor=[0.5 0.5 0.5 1.0]  GraphicAmbientColor=[0.15 0.15 0.15 1.0]  GraphicEmissiveColor=[0.0 0.0 0.0 1.0]  GraphicShininess=75  GraphicOpacity=1.0
  Alpha : Outport
  Theta : Outport  Port=2
  dTheta : Outport  Port=3
  wires:
  PS-Simulink Converter2/1 -> dTheta/1
  PS-Simulink Converter1/1 -> Theta/1
  PS-Simulink Converter/1 -> Sum2/1
  Sum2/1 -> Sum/1
  Constant1/1 -> Sum2/2
  Sum/1 -> Alpha/1
  Constant/1 -> Sum/2
  Torque/1 -> Simulink-PS Converter/1
  connections:
  Revolute Joint/RConn3 -- PS-Simulink Converter2/LConn1
  Rigid Transform5/RConn1 -- Rigid Transform2/LConn1
  Revolute Joint/LConn2 -- Simulink-PS Converter/RConn1
  Mechanism Configuration/RConn1 -- Solver Configuration/RConn1 -- Rigid Transform/LConn1 -- World Frame/RConn1
  PS-Simulink Converter/LConn1 -- Revolute Joint2/RConn2
  Rigid Transform2/RConn1 -- Pendulum/LConn1
  Rigid Transform8/RConn1 -- Rod/RConn1 -- Rigid Transform5/LConn1
  Revolute Joint/RConn1 -- Rigid Transform7/LConn1
  Encoder/LConn1 -- Rigid Transform4/LConn1 -- Rigid Transform7/RConn1
  Revolute Joint/LConn1 -- Rigid Transform3/LConn1 -- Rigid Transform1/RConn1
  scale/RConn1 -- Rigid Transform3/RConn1
  Rigid Transform4/RConn1 -- Revolute Joint2/LConn1
  Base/RConn1 -- Rigid Transform1/LConn1 -- Rigid Transform/RConn1
  Rigid Transform8/LConn1 -- Rotation Indicator/LConn1 -- Revolute Joint2/RConn1
  PS-Simulink Converter1/LConn1 -- Revolute Joint/RConn2

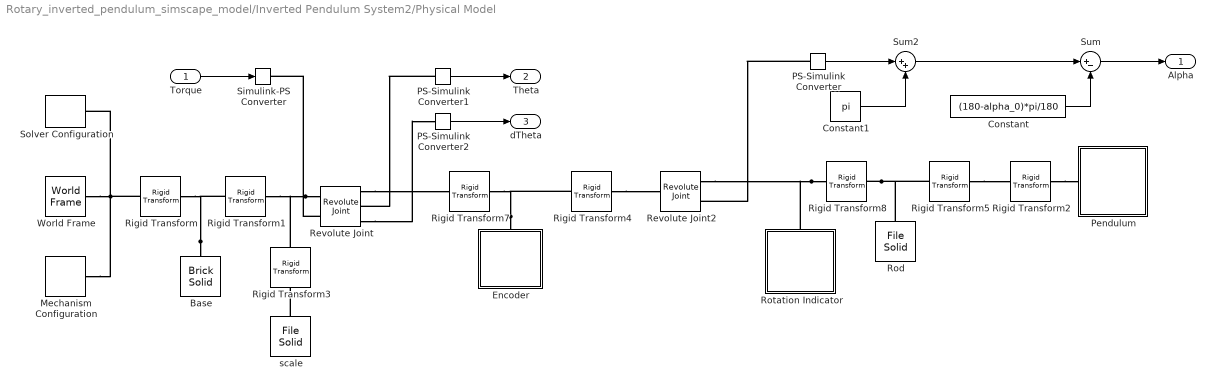
== system Rotary_inverted_pendulum_simscape_model/Inverted Pendulum System2/Physical Model ==
  Torque : Inport
  Base : sm_lib/Body Elements/Brick Solid  GraphicAmbientColor=[0.15 0.15 0.15 1.0]  BasedOnType=Density  BrickDimensions=[1 1 1]*base_size  BrickDimensionUnits=cm  CenterOfMass=[0 0 0]  CenterOfMassUnits=m  GraphicDiffuseColor=[0.4 0.4 0.4]  Density=1000  DensityUnits=kg/m^3  DoExposeReferenceFrame=on  GraphicEmissiveColor=[0.0 0.0 0.0 1.0]  ExportEntireGeometry=off  SerializedFrames=<Frames/>  MarkerShape=Sphere  MarkerSize=10  GraphicType=FromGeometry  InertiaType=CalculateFromGeometry  Mass=1  MassUnits=kg  MomentsOfInertia=[1 1 1]  MomentsOfInertiaUnits=kg*m^2  GraphicOpacity=1.0  ProductsOfInertia=[0 0 0]  ProductsOfInertiaUnits=kg*m^2  GraphicShininess=75  GraphicSpecularColor=[0.5 0.5 0.5 1.0]  GraphicVisPropType=SimpleVisualProperties
  Constant : Constant  Value=(180-alpha_0)*pi/180
  Constant1 : Constant  Value=pi
  Encoder : Subsystem
  Mechanism Configuration : sm_lib/Utilities/Mechanism Configuration  UniformGravity=Constant  GravityVector=[0 0 -9.80665]  GravityUnits=m/s^2  LinearizationDelta=0.001
  PS-Simulink Converter : nesl_utility/PS-Simulink Converter  PhysicalDomain=network_engine_domain  SubClassName=ps_output  LeftPortType=input  RightPortType=output  PseudoPeriodic=off  Frequencies=[]  Unit=inherit  AffineConversion=off
  PS-Simulink Converter1 : nesl_utility/PS-Simulink Converter  PhysicalDomain=network_engine_domain  SubClassName=ps_output  LeftPortType=input  RightPortType=output  PseudoPeriodic=off  Frequencies=[]  Unit=inherit  AffineConversion=off
  PS-Simulink Converter2 : nesl_utility/PS-Simulink Converter  PhysicalDomain=network_engine_domain  SubClassName=ps_output  LeftPortType=input  RightPortType=output  PseudoPeriodic=off  Frequencies=[]  Unit=inherit  AffineConversion=off
  Pendulum : Subsystem
  Revolute Joint : sm_lib/Joints/Revolute Joint  JointMode=Normal  SenseConstraintForce=off  SenseConstraintForceX=off  SenseConstraintForceY=off  SenseConstraintForceZ=off  SenseConstraintTorque=off  SenseConstraintTorqueX=off  SenseConstraintTorqueY=off  SenseConstraintTorqueZ=off  SenseTotalForce=off  SenseTotalForceX=off  SenseTotalForceY=off  SenseTotalForceZ=off  SenseTotalTorque=off  SenseTotalTorqueX=off  SenseTotalTorqueY=off  SenseTotalTorqueZ=off  CompositeWrenchDir=FollowerOnBase  CompositeWrenchFrame=BaseFrame  EquilibriumPosition=0  EquilibriumPositionUnits=deg  SpringStiffness=0  SpringStiffnessUnits=N*m/deg  DampingCoefficient=D_r  DampingCoefficientUnits=N*m/(rad/s)  TorqueActuationMode=InputTorque  MotionActuationMode=ComputedMotion  SensePosition=on  SenseVelocity=on  SenseAcceleration=off  SenseTorqueForce=off  SenseLowerLimitTorqueForce=off  SenseUpperLimitTorqueForce=off  LowerLimitSpecify=off  LowerLimitBound=-90  LowerLimitBoundUnits=deg  LowerLimitStiffness=1e4  LowerLimitStiffnessUnits=N*m/deg  LowerLimitDamping=10  LowerLimitDampingUnits=N*m/(deg/s)  LowerLimitTransitionRegionWidth=0.1  LowerLimitTransitionRegionWidthUnits=deg  UpperLimitSpecify=off  UpperLimitBound=90  UpperLimitBoundUnits=deg  UpperLimitStiffness=1e4  UpperLimitStiffnessUnits=N*m/deg  UpperLimitDamping=10  UpperLimitDampingUnits=N*m/(deg/s)  UpperLimitTransitionRegionWidth=0.1  UpperLimitTransitionRegionWidthUnits=deg  PositionTargetSpecify=off  PositionTargetPriority=High  PositionTargetValue=0  PositionTargetValueUnits=deg  VelocityTargetSpecify=off  VelocityTargetPriority=High  VelocityTargetValue=0  VelocityTargetValueUnits=deg/s
  Revolute Joint2 : sm_lib/Joints/Revolute Joint  JointMode=Normal  SenseConstraintForce=off  SenseConstraintForceX=off  SenseConstraintForceY=off  SenseConstraintForceZ=off  SenseConstraintTorque=off  SenseConstraintTorqueX=off  SenseConstraintTorqueY=off  SenseConstraintTorqueZ=off  SenseTotalForce=off  SenseTotalForceX=off  SenseTotalForceY=off  SenseTotalForceZ=off  SenseTotalTorque=off  SenseTotalTorqueX=off  SenseTotalTorqueY=off  SenseTotalTorqueZ=off  CompositeWrenchDir=FollowerOnBase  CompositeWrenchFrame=BaseFrame  EquilibriumPosition=0  EquilibriumPositionUnits=deg  SpringStiffness=0  SpringStiffnessUnits=N*m/deg  DampingCoefficient=D_p  DampingCoefficientUnits=N*m/(rad/s)  TorqueActuationMode=NoTorque  MotionActuationMode=ComputedMotion  SensePosition=on  SenseVelocity=off  SenseAcceleration=off  SenseTorqueForce=off  SenseLowerLimitTorqueForce=off  SenseUpperLimitTorqueForce=off  LowerLimitSpecify=off  LowerLimitBound=-90  LowerLimitBoundUnits=deg  LowerLimitStiffness=1e4  LowerLimitStiffnessUnits=N*m/deg  LowerLimitDamping=10  LowerLimitDampingUnits=N*m/(deg/s)  LowerLimitTransitionRegionWidth=0.1  LowerLimitTransitionRegionWidthUnits=deg  UpperLimitSpecify=off  UpperLimitBound=90  UpperLimitBoundUnits=deg  UpperLimitStiffness=1e4  UpperLimitStiffnessUnits=N*m/deg  UpperLimitDamping=10  UpperLimitDampingUnits=N*m/(deg/s)  UpperLimitTransitionRegionWidth=0.1  UpperLimitTransitionRegionWidthUnits=deg  PositionTargetSpecify=off  PositionTargetPriority=High  PositionTargetValue=0  PositionTargetValueUnits=deg  VelocityTargetSpecify=off  VelocityTargetPriority=High  VelocityTargetValue=0  VelocityTargetValueUnits=deg/s
  Rigid Transform : sm_lib/Frames and Transforms/Rigid Transform  TranslationMethod=None  TranslationStandardOffset=0  TranslationLengthUnit=m  TranslationStandardAxis=+Z  TranslationCartesianOffset=[0 0 0]  TranslationROffset=0  TranslationROffsetUnits=m  TranslationZOffset=0  TranslationZOffsetUnits=m  TranslationThetaOffset=0  TranslationThetaOffsetUnits=deg  RotationMethod=None  RotationAngleUnits=deg  RotationStandardAxis=+Z  RotationAngle=0.0  RotationArbitraryAxis=[0 0 1]  FollAlignAxisA=+X  BaseAlignAxisA=+Y  FollAlignAxisB=+Y  BaseAlignAxisB=+Z  RotationSequenceAxes=FollowerAxes  RotationSequence=XYX  RotationSequenceAngles=[0 0 0]  RotationSequenceAnglesUnits=deg  RotationMatrix=[1 0 0; 0 1 0; 0 0 1]
  Rigid Transform1 : sm_lib/Frames and Transforms/Rigid Transform  TranslationMethod=Cartesian  TranslationStandardOffset=0  TranslationLengthUnit=cm  TranslationStandardAxis=+Z  TranslationCartesianOffset=[0 0 rt1]  TranslationROffset=0  TranslationROffsetUnits=m  TranslationZOffset=0  TranslationZOffsetUnits=m  TranslationThetaOffset=0  TranslationThetaOffsetUnits=deg  RotationMethod=None  RotationAngleUnits=deg  RotationStandardAxis=+Y  RotationAngle=90  RotationArbitraryAxis=[0 0 1]  FollAlignAxisA=+X  BaseAlignAxisA=+Y  FollAlignAxisB=+Y  BaseAlignAxisB=+Z  RotationSequenceAxes=FollowerAxes  RotationSequence=XYX  RotationSequenceAngles=[0 0 0]  RotationSequenceAnglesUnits=deg  RotationMatrix=[1 0 0; 0 1 0; 0 0 1]
  Rigid Transform2 : sm_lib/Frames and Transforms/Rigid Transform  TranslationMethod=Cartesian  TranslationStandardOffset=0  TranslationLengthUnit=cm  TranslationStandardAxis=+Z  TranslationCartesianOffset=[0 0 rt2]  TranslationROffset=0  TranslationROffsetUnits=m  TranslationZOffset=0  TranslationZOffsetUnits=m  TranslationThetaOffset=0  TranslationThetaOffsetUnits=deg  RotationMethod=None  RotationAngleUnits=deg  RotationStandardAxis=+Y  RotationAngle=90  RotationArbitraryAxis=[0 0 1]  FollAlignAxisA=+X  BaseAlignAxisA=+Y  FollAlignAxisB=+Y  BaseAlignAxisB=+Z  RotationSequenceAxes=FollowerAxes  RotationSequence=XYX  RotationSequenceAngles=[0 0 0]  RotationSequenceAnglesUnits=deg  RotationMatrix=[1 0 0; 0 1 0; 0 0 1]
  Rigid Transform3 : sm_lib/Frames and Transforms/Rigid Transform  TranslationMethod=None  TranslationStandardOffset=0  TranslationLengthUnit=cm  TranslationStandardAxis=+Z  TranslationCartesianOffset=[0 0 rt1]  TranslationROffset=0  TranslationROffsetUnits=m  TranslationZOffset=0  TranslationZOffsetUnits=m  TranslationThetaOffset=0  TranslationThetaOffsetUnits=deg  RotationMethod=RotationSequence  RotationAngleUnits=deg  RotationStandardAxis=+X  RotationAngle=90  RotationArbitraryAxis=[0 0 1]  FollAlignAxisA=+X  BaseAlignAxisA=+Y  FollAlignAxisB=+Y  BaseAlignAxisB=+Z  RotationSequenceAxes=FollowerAxes  RotationSequence=XYX  RotationSequenceAngles=[90 -90 0]  RotationSequenceAnglesUnits=deg  RotationMatrix=[1 0 0; 0 1 0; 0 0 1]
  Rigid Transform4 : sm_lib/Frames and Transforms/Rigid Transform  TranslationMethod=Cartesian  TranslationStandardOffset=0  TranslationLengthUnit=cm  TranslationStandardAxis=+Z  TranslationCartesianOffset=[-1.3 1 0]  TranslationROffset=0  TranslationROffsetUnits=m  TranslationZOffset=0  TranslationZOffsetUnits=m  TranslationThetaOffset=0  TranslationThetaOffsetUnits=deg  RotationMethod=StandardAxis  RotationAngleUnits=deg  RotationStandardAxis=+Y  RotationAngle=90  RotationArbitraryAxis=[0 0 1]  FollAlignAxisA=+X  BaseAlignAxisA=+Y  FollAlignAxisB=+Y  BaseAlignAxisB=+Z  RotationSequenceAxes=FollowerAxes  RotationSequence=XYX  RotationSequenceAngles=[0 0 0]  RotationSequenceAnglesUnits=deg  RotationMatrix=[1 0 0; 0 1 0; 0 0 1]
  Rigid Transform5 : sm_lib/Frames and Transforms/Rigid Transform  TranslationMethod=None  TranslationStandardOffset=0  TranslationLengthUnit=cm  TranslationStandardAxis=+Z  TranslationCartesianOffset=[0 0 rt2]  TranslationROffset=0  TranslationROffsetUnits=m  TranslationZOffset=0  TranslationZOffsetUnits=m  TranslationThetaOffset=0  TranslationThetaOffsetUnits=deg  RotationMethod=StandardAxis  RotationAngleUnits=deg  RotationStandardAxis=+Y  RotationAngle=90  RotationArbitraryAxis=[0 0 1]  FollAlignAxisA=+X  BaseAlignAxisA=+Y  FollAlignAxisB=+Y  BaseAlignAxisB=+Z  RotationSequenceAxes=FollowerAxes  RotationSequence=XYX  RotationSequenceAngles=[0 0 0]  RotationSequenceAnglesUnits=deg  RotationMatrix=[1 0 0; 0 1 0; 0 0 1]
  Rigid Transform7 : sm_lib/Frames and Transforms/Rigid Transform  TranslationMethod=Cartesian  TranslationStandardOffset=0  TranslationLengthUnit=cm  TranslationStandardAxis=+Z  TranslationCartesianOffset=[0 0 0.5]  TranslationROffset=0  TranslationROffsetUnits=m  TranslationZOffset=0  TranslationZOffsetUnits=m  TranslationThetaOffset=0  TranslationThetaOffsetUnits=deg  RotationMethod=StandardAxis  RotationAngleUnits=deg  RotationStandardAxis=+X  RotationAngle=90  RotationArbitraryAxis=[0 0 1]  FollAlignAxisA=+X  BaseAlignAxisA=+Y  FollAlignAxisB=+Y  BaseAlignAxisB=+Z  RotationSequenceAxes=FollowerAxes  RotationSequence=XYX  RotationSequenceAngles=[0 0 0]  RotationSequenceAnglesUnits=deg  RotationMatrix=[1 0 0; 0 1 0; 0 0 1]
  Rigid Transform8 : sm_lib/Frames and Transforms/Rigid Transform  TranslationMethod=None  TranslationStandardOffset=0  TranslationLengthUnit=cm  TranslationStandardAxis=+Z  TranslationCartesianOffset=[-1.3 1 0]  TranslationROffset=0  TranslationROffsetUnits=m  TranslationZOffset=0  TranslationZOffsetUnits=m  TranslationThetaOffset=0  TranslationThetaOffsetUnits=deg  RotationMethod=StandardAxis  RotationAngleUnits=deg  RotationStandardAxis=+Y  RotationAngle=-90  RotationArbitraryAxis=[0 0 1]  FollAlignAxisA=+X  BaseAlignAxisA=+Y  FollAlignAxisB=+Y  BaseAlignAxisB=+Z  RotationSequenceAxes=FollowerAxes  RotationSequence=XYX  RotationSequenceAngles=[0 0 0]  RotationSequenceAnglesUnits=deg  RotationMatrix=[1 0 0; 0 1 0; 0 0 1]
  Rod : sm_lib/Body Elements/File Solid  ExtGeomFileName=step_rod.STEP  UnitType=FromFile  ExtGeomFileUnits=cm  StepReaderType=HEX  ExportEntireGeometry=off  InertiaType=CalculateFromGeometry  Mass=rod_mass  MassUnits=kg  CenterOfMass=[0 0 0]  CenterOfMassUnits=m  MomentsOfInertia=[1 1 1]  MomentsOfInertiaUnits=kg*m^2  ProductsOfInertia=[0 0 0]  ProductsOfInertiaUnits=kg*m^2  BasedOnType=Mass  Density=1000  DensityUnits=kg/m^3  DoExposeReferenceFrame=on  SerializedFrames=<Frames/>  GraphicType=FromGeometry  MarkerShape=Frame  MarkerSize=10  GraphicVisPropType=FromFileVisualProperties  GraphicDiffuseColor=[0.5 0.5 0.5]  GraphicSpecularColor=[0.5 0.5 0.5 1.0]  GraphicAmbientColor=[0.15 0.15 0.15 1.0]  GraphicEmissiveColor=[0.0 0.0 0.0 1.0]  GraphicShininess=75  GraphicOpacity=1.0
  Rotation Indicator : Subsystem
  Simulink-PS Converter : nesl_utility/Simulink-PS Converter  PhysicalDomain=network_engine_domain  SubClassName=ps_input  LeftPortType=input  RightPortType=output  PseudoPeriodic=off  Frequencies=[]  NoiseDistribution=none  NoiseParameters=[]  Unit=1  AffineConversion=off  FilteringAndDerivatives=provide  SimscapeFilterOrder=1  InputFilterTimeConstant=0.001  UdotUserProvided=0
  Solver Configuration : nesl_utility/Solver Configuration  PhysicalDomain=network_engine_domain  SubClassName=solver  LeftPortType=input  RightPortType=generic  Tones=[]  Harmonics=[]  SimulateNoise=off  Profile=off  UseLocalSampling=off  EnableSwitchedLinearOptims=on  FrequencyDomain=off  UseCCode=off  RelTol=0.001  AbsTol=1e-06  MinStep=1e-09  ToWorkspace=off  RevertToSquareIcSolve=off  NumHomotopyIterations=100  PhasorMode=off  PhasorModeNumHarmonics=1  DoDC=off  ResidualTolerance=1e-09  UseLocalSolver=off  LocalSolverChoice=NE_BACKWARD_EULER_ADVANCER  LocalSolverSampleTime=0.001  DoFixedCost=off  MaxNonlinIter=3  MaxModeIter=2  LinearAlgebra=Sparse  EquationFormulation=NE_TIME_EF  DelaysMemoryBudget=1024  AutomaticFiltering=on  FilteringTimeConstant=0.001  PartitionStorageMethod=AS_NEEDED  PartitionMemoryBudget=1024  PartitionMethod=FAST
  Sum : Sum  Inputs=|+-
  Sum2 : Sum  Inputs=|++
  World Frame : sm_lib/Frames and Transforms/World Frame
  scale : sm_lib/Body Elements/File Solid  ExtGeomFileName=step_angles.STEP  UnitType=FromFile  ExtGeomFileUnits=cm  StepReaderType=HEX  ExportEntireGeometry=off  InertiaType=CalculateFromGeometry  Mass=rod_mass  MassUnits=kg  CenterOfMass=[0 0 0]  CenterOfMassUnits=m  MomentsOfInertia=[1 1 1]  MomentsOfInertiaUnits=kg*m^2  ProductsOfInertia=[0 0 0]  ProductsOfInertiaUnits=kg*m^2  BasedOnType=Mass  Density=1000  DensityUnits=kg/m^3  DoExposeReferenceFrame=on  SerializedFrames=<Frames/>  GraphicType=FromGeometry  MarkerShape=Frame  MarkerSize=10  GraphicVisPropType=SimpleVisualProperties  GraphicDiffuseColor=[1.0 1.0 1.0]  GraphicSpecularColor=[0.5 0.5 0.5 1.0]  GraphicAmbientColor=[0.15 0.15 0.15 1.0]  GraphicEmissiveColor=[0.0 0.0 0.0 1.0]  GraphicShininess=75  GraphicOpacity=1.0
  Alpha : Outport
  Theta : Outport  Port=2
  dTheta : Outport  Port=3
  wires:
  PS-Simulink Converter2/1 -> dTheta/1
  PS-Simulink Converter1/1 -> Theta/1
  PS-Simulink Converter/1 -> Sum2/1
  Sum2/1 -> Sum/1
  Constant1/1 -> Sum2/2
  Sum/1 -> Alpha/1
  Constant/1 -> Sum/2
  Torque/1 -> Simulink-PS Converter/1
  connections:
  Revolute Joint/RConn3 -- PS-Simulink Converter2/LConn1
  Rigid Transform5/RConn1 -- Rigid Transform2/LConn1
  Revolute Joint/LConn2 -- Simulink-PS Converter/RConn1
  Mechanism Configuration/RConn1 -- Solver Configuration/RConn1 -- Rigid Transform/LConn1 -- World Frame/RConn1
  PS-Simulink Converter/LConn1 -- Revolute Joint2/RConn2
  Rigid Transform2/RConn1 -- Pendulum/LConn1
  Rigid Transform8/RConn1 -- Rod/RConn1 -- Rigid Transform5/LConn1
  Revolute Joint/RConn1 -- Rigid Transform7/LConn1
  Encoder/LConn1 -- Rigid Transform4/LConn1 -- Rigid Transform7/RConn1
  Revolute Joint/LConn1 -- Rigid Transform3/LConn1 -- Rigid Transform1/RConn1
  scale/RConn1 -- Rigid Transform3/RConn1
  Rigid Transform4/RConn1 -- Revolute Joint2/LConn1
  Base/RConn1 -- Rigid Transform1/LConn1 -- Rigid Transform/RConn1
  Rigid Transform8/LConn1 -- Rotation Indicator/LConn1 -- Revolute Joint2/RConn1
  PS-Simulink Converter1/LConn1 -- Revolute Joint/RConn2
